simulink model "SMC_model"  (R2026b)
settings: Solver=ode23tb  StopTime=0.2  MaxStep=1e-5  AbsTol=1e-3
settings Model: Creator=flyfoar  LastModifiedBy=flyfoar

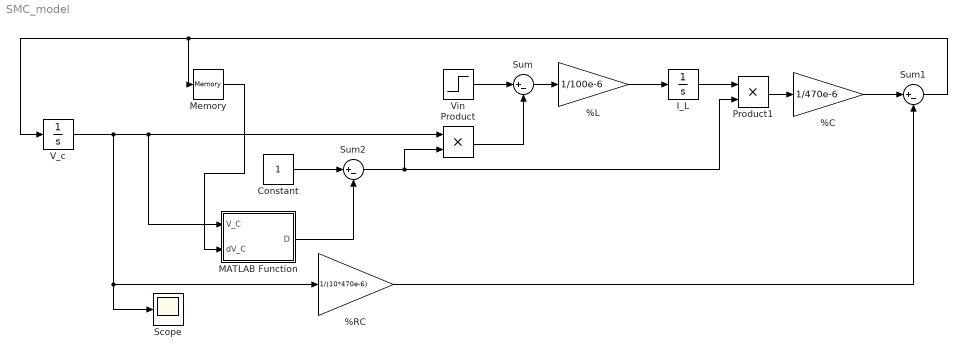
== system SMC_model ==
  %C : Gain  Gain=1/470e-6
  %L : Gain  Gain=1/100e-6
  %RC : Gain  Gain=1/(10*470e-6)
  Constant : Constant
  I_L : Integrator
  MATLAB Function : MATLAB Function  TreatAsAtomicUnit=on
  Memory : Memory
  Product : Product
  Product1 : Product
  Scope : Scope
      settings: ActiveDisplayYMinimum=13.343388206925111  ActiveDisplayYMaximum=41.402550771728556
  Sum : Sum  Inputs=|+-
  Sum1 : Sum  Inputs=|+-
  Sum2 : Sum  Inputs=|+-
  V_c : Integrator
  Vin : Step  Time=0.025  InitialValue=12  FinalValue=9  SampleTime=0
  wires:
  V_c/1 -> Scope/1, %RC/1, Product/1, MATLAB Function/1(V_C)
  %L/1 -> I_L/1
  Sum1/1 -> Memory/1, V_c/1
  Product1/1 -> %C/1
  Constant/1 -> Sum2/1
  MATLAB Function/1(D) -> Sum2/2
  Sum2/1 -> Product/2, Product1/2
  %RC/1 -> Sum1/2
  %C/1 -> Sum1/1
  Vin/1 -> Sum/1
  Product/1 -> Sum/2
  Sum/1 -> %L/1
  I_L/1 -> Product1/1
  Memory/1 -> MATLAB Function/2(dV_C)

== matlab function SMC_model/MATLAB Function ==
  data: V_C input; D output; dV_C input
function D = smc(V_C, dV_C)
V_ref = 22.5;
lambda = 0.001;
phi = 2;

e = V_C - V_ref;
s = e + lambda * dV_C;

if s > phi
    D = 0.1;
elseif s < -phi
    D = 0.9;
else
    D = 0.5 - (s / (2*phi)) * 0.4;
end
end
